simulink model "ekf_mr2006b_211126"  (R2026a)
settings: Solver=FixedStepDiscrete  StopTime=60.000000  FixedStep=1/1666000
PreLoadFcn:
  | addpath(genpath('/Users/danielappel/Developer/euromotion-tec/Matlab/ekf_design'));
InitFcn:
  | addpath(genpath('/Users/danielappel/Developer/euromotion-tec/Matlab/ekf_design'));
undefined symbols (not defined in the file or in its folder): ekf_course, ekf_p, ekf_tr
settings Model: ExtModeTrigDuration=10000  Creator=danielappel  LastModifiedBy=danielappel
settings DebuggingCC: AlgebraicLoopMsg=error

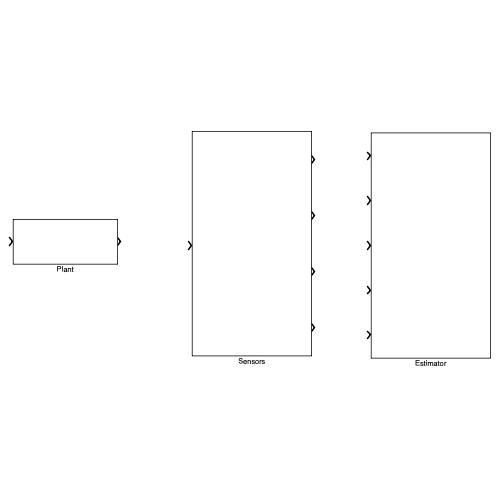
[thumbnail: Simulink's stored preview of the top-level diagram]
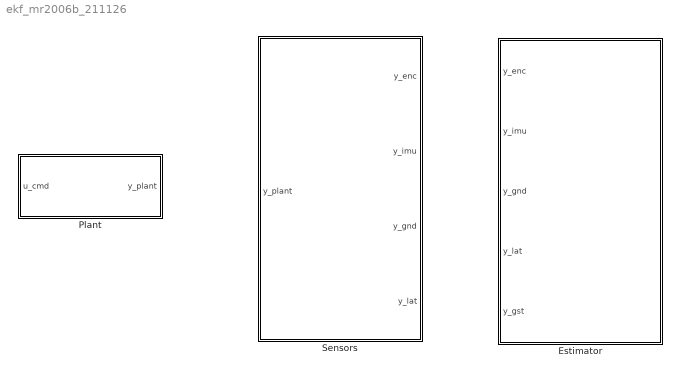
== system ekf_mr2006b_211126 ==
  Estimator : Subsystem
  Plant : Subsystem  TreatAsAtomicUnit=on  SystemSampleTime=1e-3
  Sensors : Subsystem

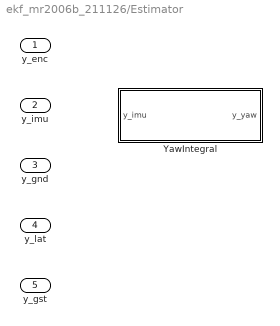
== system ekf_mr2006b_211126/Estimator ==
  y_enc : Inport
  y_imu : Inport  Port=2
  y_gnd : Inport  Port=3
  y_lat : Inport  Port=4
  y_gst : Inport  Port=5
  YawIntegral : Subsystem  TreatAsAtomicUnit=on  SystemSampleTime=1e-3

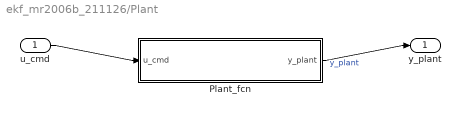
== system ekf_mr2006b_211126/Plant ==
  u_cmd : Inport
  Plant_fcn : MATLAB Function  TreatAsAtomicUnit=on
  y_plant : Outport
  wires:
  u_cmd/1 -> Plant_fcn/1(u_cmd)
  Plant_fcn/1(y_plant) -> y_plant/1  "y_plant"

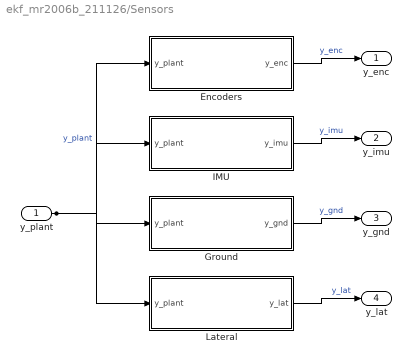
== system ekf_mr2006b_211126/Sensors ==
  y_plant : Inport
  Encoders : Subsystem  TreatAsAtomicUnit=on  SystemSampleTime=1e-3
  Ground : Subsystem  TreatAsAtomicUnit=on  SystemSampleTime=1e-3
  IMU : Subsystem  TreatAsAtomicUnit=on  SystemSampleTime=[1/833 1/1666000]
  Lateral : Subsystem  TreatAsAtomicUnit=on  SystemSampleTime=1e-3
  y_enc : Outport
  y_imu : Outport  Port=2
  y_gnd : Outport  Port=3
  y_lat : Outport  Port=4
  wires:
  y_plant/1 -> Encoders/1(y_plant), IMU/1(y_plant), Ground/1(y_plant), Lateral/1(y_plant)  "y_plant"
  Encoders/1(y_enc) -> y_enc/1  "y_enc"
  IMU/1(y_imu) -> y_imu/1  "y_imu"
  Ground/1(y_gnd) -> y_gnd/1  "y_gnd"
  Lateral/1(y_lat) -> y_lat/1  "y_lat"

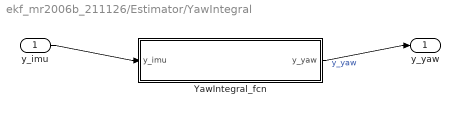
== system ekf_mr2006b_211126/Estimator/YawIntegral ==
  y_imu : Inport
  YawIntegral_fcn : MATLAB Function  TreatAsAtomicUnit=on
  y_yaw : Outport
  wires:
  y_imu/1 -> YawIntegral_fcn/1(y_imu)
  YawIntegral_fcn/1(y_yaw) -> y_yaw/1  "y_yaw"

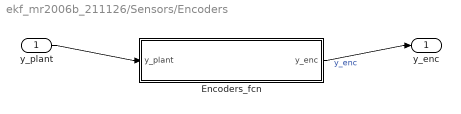
== system ekf_mr2006b_211126/Sensors/Encoders ==
  y_plant : Inport
  Encoders_fcn : MATLAB Function  TreatAsAtomicUnit=on
  y_enc : Outport
  wires:
  y_plant/1 -> Encoders_fcn/1(y_plant)
  Encoders_fcn/1(y_enc) -> y_enc/1  "y_enc"

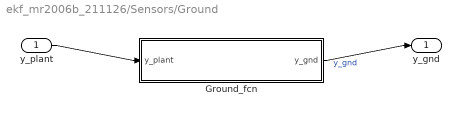
== system ekf_mr2006b_211126/Sensors/Ground ==
  y_plant : Inport
  Ground_fcn : MATLAB Function  TreatAsAtomicUnit=on
  y_gnd : Outport
  wires:
  y_plant/1 -> Ground_fcn/1(y_plant)
  Ground_fcn/1(y_gnd) -> y_gnd/1  "y_gnd"

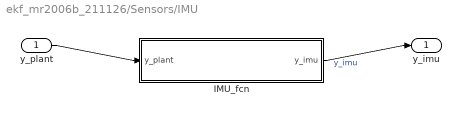
== system ekf_mr2006b_211126/Sensors/IMU ==
  y_plant : Inport
  IMU_fcn : MATLAB Function  TreatAsAtomicUnit=on
  y_imu : Outport
  wires:
  y_plant/1 -> IMU_fcn/1(y_plant)
  IMU_fcn/1(y_imu) -> y_imu/1  "y_imu"

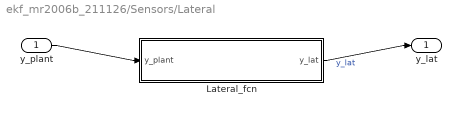
== system ekf_mr2006b_211126/Sensors/Lateral ==
  y_plant : Inport
  Lateral_fcn : MATLAB Function  TreatAsAtomicUnit=on
  y_lat : Outport
  wires:
  y_plant/1 -> Lateral_fcn/1(y_plant)
  Lateral_fcn/1(y_lat) -> y_lat/1  "y_lat"

== matlab function ekf_mr2006b_211126/Sensors/Encoders/Encoders_fcn ==
  data: y_plant input; y_enc output; ekf_p parameter
function y_enc = fcn(y_plant, ekf_p)
%#codegen
y_enc = sim_enc_step(y_plant, ekf_p);

== matlab function ekf_mr2006b_211126/Plant/Plant_fcn ==
  data: u_cmd input; y_plant output; ekf_tr parameter; ekf_course parameter
function y_plant = fcn(u_cmd, ekf_tr, ekf_course)
%#codegen
persistent st
if isempty(st)
    st = sim_plant_init(ekf_tr, ekf_course);
end
[st, y_plant] = sim_plant_step(st, u_cmd, ekf_tr);

== matlab function ekf_mr2006b_211126/Sensors/IMU/IMU_fcn ==
  data: y_plant input; y_imu output; ekf_tr parameter
function y_imu = fcn(y_plant, ekf_tr)
%#codegen
persistent st
if isempty(st)
    st = sim_imu_init(ekf_tr);
end
[st, y_imu] = sim_imu_step(st, y_plant, ekf_tr);

== matlab function ekf_mr2006b_211126/Sensors/Ground/Ground_fcn ==
  data: y_plant input; y_gnd output; ekf_tr parameter; ekf_course parameter; ekf_p parameter
function y_gnd = fcn(y_plant, ekf_tr, ekf_course, ekf_p)
%#codegen
persistent st
if isempty(st)
    st = sim_gnd_init(ekf_tr, ekf_course, ekf_p);
end
[st, y_gnd] = sim_gnd_step(st, y_plant, ekf_tr, ekf_course, ekf_p);

== matlab function ekf_mr2006b_211126/Sensors/Lateral/Lateral_fcn ==
  data: y_plant input; y_lat output; ekf_tr parameter; ekf_course parameter; ekf_p parameter
function y_lat = fcn(y_plant, ekf_tr, ekf_course, ekf_p)
%#codegen
persistent st
if isempty(st)
    st = sim_lat_init(ekf_tr, ekf_p);
end
[st, y_lat] = sim_lat_step(st, y_plant, ekf_tr, ekf_course, ekf_p);

== matlab function ekf_mr2006b_211126/Estimator/YawIntegral/YawIntegral_fcn ==
  data: y_imu input; y_yaw output; ekf_pc parameter
function y_yaw = fcn(y_imu, ekf_pc)
%#codegen
persistent st
if isempty(st)
    st = sim_yaw_init(ekf_pc);
end
[st, y_yaw] = sim_yaw_step(st, y_imu, ekf_pc);
